simulink model "mu_nonlinear_sim"  (R2026a)
settings: Solver=VariableStepAuto
InitFcn:
  | seaDir=fileparts(get_param(bdroot,'FileName'));if isfile(fullfile(seaDir,'..','collaudo_simulink.m')),addpath(fullfile(seaDir,'..'));else,addpath(fullfile(seaDir,'..','..','File_di_Funzioni_Progetto-Accorpati'));end;collaudo_simulink(bdroot);
undefined symbols (not defined in the file): taubar, xbar
libraries: cstblocks_lti x3
settings Model: Creator=rebec  LastModifiedBy=rebec

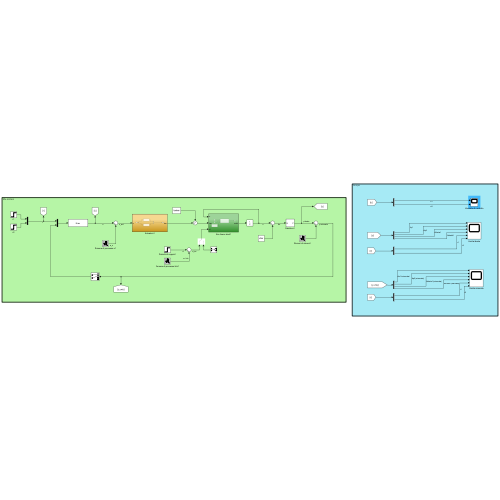
[thumbnail: Simulink's stored preview of the top-level diagram]
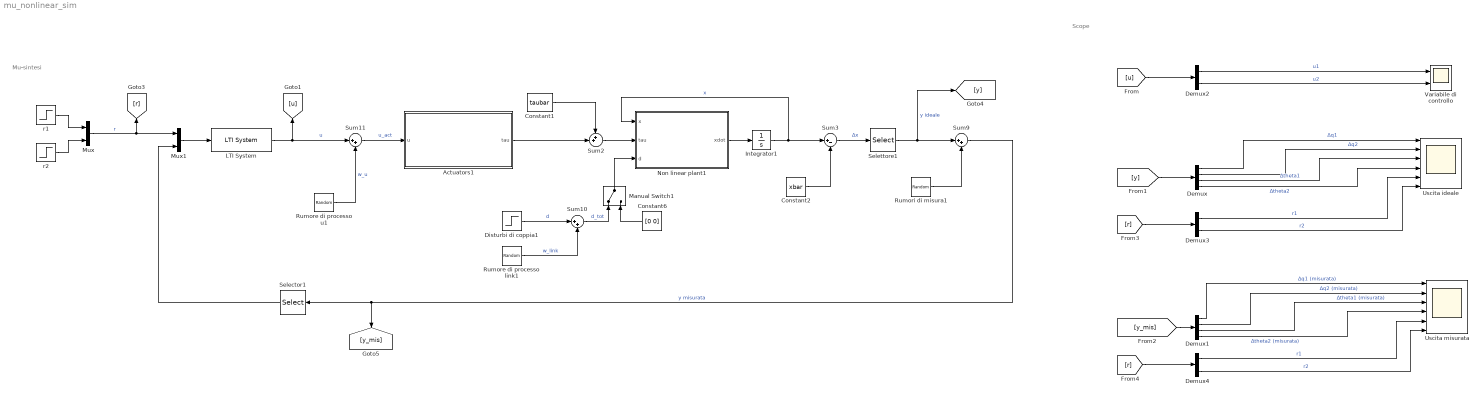
== system mu_nonlinear_sim ==
  note: Scope
  note: Mu-sintesi
  Actuators1 : Subsystem
  Constant1 : Constant  Value=taubar
  Constant2 : Constant  Value=xbar
  Constant6 : Constant  Value=[0 0]
  Demux : Demux
  Demux1 : Demux
  Demux2 : Demux  Outputs=2
  Demux3 : Demux  Outputs=2
  Demux4 : Demux  Outputs=2
  Disturbi di coppia1 : Step  Time=[1 1]  InitialValue=[0 0]  FinalValue=[0.5 0]  SampleTime=0
  Integrator1 : Integrator  InitialCondition=xbar
  LTI System : cstblocks_lti/LTI System  sys=Kmu  IC=[]  PadeOrder=0
      settings: LibrarySourceBlock=cstblocks/LTI System
  Manual Switch1 : ManualSwitch
  Mux : Mux  Inputs=2
  Mux1 : Mux  Inputs=2
  Non linear plant1 : Subsystem
  Rumore di processo link1 : RandomNumber  Mean=[0 0]  Variance=[0.01 0.01]  Seed=20260826  SampleTime=0.002
  Rumore di processo u1 : RandomNumber  Mean=[0 0]  Variance=[0.01 0.01]  Seed=20260826  SampleTime=0.002
  Rumori di misura1 : RandomNumber  Mean=[0 0 0 0]  Variance=[(0.05*pi/180)^2 (0.05*pi/180)^2 (0.05*pi/180)^2 (0.05*pi/180)^2]  Seed=20260826  SampleTime=0.002
  Selector1 : Selector  InputPortWidth=4  IndexOptions=Index vector (dialog)  Indices=[1 2]  OutputSizes=1
  Selettore1 : Selector  InputPortWidth=8  IndexOptions=Index vector (dialog)  Indices=[1 2 5 6]  OutputSizes=1
  Sum10 : Sum  Inputs=|++
  Sum11 : Sum  Inputs=|++
  Sum2 : Sum  Inputs=++|
  Sum3 : Sum  Inputs=|+-
  Sum9 : Sum  Inputs=|++
  Uscita ideale : Scope  NumInputPorts=6
      settings: Title=Uscita ideale (mu NL)  ActiveDisplayYMinimum=-0.088271118920575181  ActiveDisplayYMaximum=0.23303114019935003  YLabel=y (rad)
  Uscita misurata : Scope  NumInputPorts=6
      settings: Title=Uscita misurata (mu NL)  ActiveDisplayYMinimum=-0.11442029066688837  ActiveDisplayYMaximum=0.16914890182413583  YLabel=y (rad)
  Variabile di controllo : Scope  NumInputPorts=2
      settings: Title=Variabili di controllo (mu NL)  ActiveDisplayYMinimum=-14.512240124873713  ActiveDisplayYMaximum=7.6680416810083489  YLabel=u (Nm)  DataLoggingVariableName=ScopeData2
  r1 : Step  FinalValue=5*pi/180  SampleTime=0
  r2 : Step  FinalValue=0  SampleTime=0
  wires:
  Manual Switch1/1 -> Non linear plant1/3(d)
  Selector1/1 -> Mux1/2
  r2/1 -> Mux/2
  Sum9/1 -> [y_mis], Selector1/1  "y misurata"
  r1/1 -> Mux/1
  Integrator1/1 -> Non linear plant1/1(x), Sum3/1  "x"
  Constant2/1 -> Sum3/2
  Sum3/1 -> Selettore1/1  "Δx"
  Sum10/1 -> Manual Switch1/1  "d_tot"
  Constant1/1 -> Sum2/1
  Sum2/1 -> Non linear plant1/2(tau)
  Constant6/1 -> Manual Switch1/2
  Sum11/1 -> Actuators1/1(u)  "u_act"
  Mux/1 -> Mux1/1, [r]  "r"
  Actuators1/1(tau) -> Sum2/2
  Rumore di processo u1/1 -> Sum11/2  "w_u"
  LTI System/1 -> Sum11/1, [u]  "u"
  Selettore1/1 -> Sum9/1, [y]  "y ideale"
  Rumore di processo link1/1 -> Sum10/2  "w_link"
  Disturbi di coppia1/1 -> Sum10/1  "d"
  Mux1/1 -> LTI System/1
  Non linear plant1/1(xdot) -> Integrator1/1
  [y_mis] -> Demux1/1
  Demux4/2 -> Uscita misurata/6  "r2"
  Demux1/4 -> Uscita misurata/4  "Δtheta2 (misurata)"
  [r] -> Demux3/1
  Demux1/2 -> Uscita misurata/2  "Δq2 (misurata)"
  Demux4/1 -> Uscita misurata/5  "r1"
  [r] -> Demux4/1
  Demux/3 -> Uscita ideale/3  "Δtheta1"
  Demux/4 -> Uscita ideale/4  "Δtheta2"
  [y] -> Demux/1
  Demux/1 -> Uscita ideale/1  "Δq1"
  Demux/2 -> Uscita ideale/2  "Δq2"
  Demux2/1 -> Variabile di controllo/1  "u1"
  Demux3/2 -> Uscita ideale/6  "r2"
  Demux1/3 -> Uscita misurata/3  "Δtheta1 (misurata)"
  Demux3/1 -> Uscita ideale/5  "r1"
  Demux2/2 -> Variabile di controllo/2  "u2"
  [u] -> Demux2/1
  Demux1/1 -> Uscita misurata/1  "Δq1 (misurata)"
  Rumori di misura1/1 -> Sum9/2

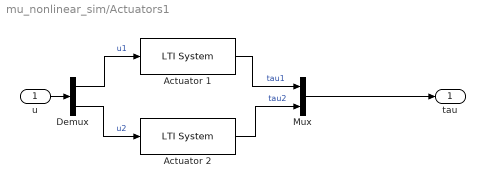
== system mu_nonlinear_sim/Actuators1 ==
  u : Inport
  Actuator 1 : cstblocks_lti/LTI System  sys=Gact  IC=[]  PadeOrder=0
      settings: LibrarySourceBlock=cstblocks/LTI System
  Actuator 2 : cstblocks_lti/LTI System  sys=Gact  IC=[]  PadeOrder=0
      settings: LibrarySourceBlock=cstblocks/LTI System
  Demux : Demux  Outputs=2
  Mux : Mux  Inputs=2
  tau : Outport
  wires:
  Actuator 2/1 -> Mux/2  "tau2"
  Demux/2 -> Actuator 2/1  "u2"
  u/1 -> Demux/1
  Demux/1 -> Actuator 1/1  "u1"
  Mux/1 -> tau/1
  Actuator 1/1 -> Mux/1  "tau1"

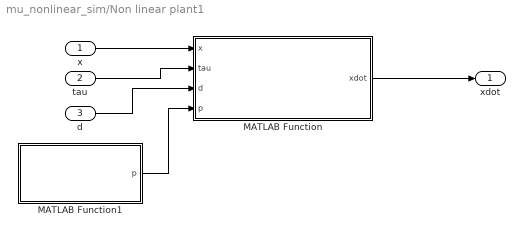
== system mu_nonlinear_sim/Non linear plant1 ==
  x : Inport
  tau : Inport  Port=2
  d : Inport  Port=3
  MATLAB Function : MATLAB Function  TreatAsAtomicUnit=on
  MATLAB Function1 : MATLAB Function  TreatAsAtomicUnit=on
  xdot : Outport
  wires:
  x/1 -> MATLAB Function/1(x)
  tau/1 -> MATLAB Function/2(tau)
  MATLAB Function/1(xdot) -> xdot/1
  MATLAB Function1/1(p) -> MATLAB Function/4(p)
  d/1 -> MATLAB Function/3(d)

== matlab function mu_nonlinear_sim/Non linear plant1/MATLAB Function ==
  data: x input; xdot output; tau input; d input; p input
function xdot = sea_nonlinear_rhs_with_link_disturbance(x, tau, d, p)
%SEA_NONLINEAR_RHS_WITH_LINK_DISTURBANCE SEA dynamics with link torque D.
%   TAU remains the motor-side input; D is an external link-side joint
%   torque entering with positive sign in the link equation.

assert(numel(x) == 8, ...
    'sea_nonlinear_rhs_with_link_disturbance:InvalidState', ...
    'The state must contain exactly eight elements.');
assert(numel(tau) == 2 && numel(d) == 2, ...
    'sea_nonlinear_rhs_with_link_disturbance:InvalidInput', ...
    'Both tau and d must contain exactly two elements.');
x = reshape(x, 8, 1);
tau = reshape(tau, 2, 1);
d = reshape(d, 2, 1);

q = x(1:2);
qdot = x(3:4);
theta = x(5:6);
thetadot = x(7:8);
M = sea_link_inertia(q, p);
C = sea_coriolis(q, qdot, p);
G = sea_gravity(q, p);
tauElastic = sea_elastic_torque(q, theta, p);

qddot = M \ (tauElastic + d - C * qdot - G);
thetaddot = p.Jm \ (tau - p.Bm * thetadot - tauElastic);
xdot = [qdot; qddot; thetadot; thetaddot];
end

== matlab function mu_nonlinear_sim/Non linear plant1/MATLAB Function1 ==
  data: p output Bus: slBus1
function p = sea_params_nominal
%SEA_PARAMS_NOMINAL Nominal mechanical parameters of the 2R SEA robot.
%   P = SEA_PARAMS_NOMINAL returns the values stated by the official
%   assignment. Matrices follow the joint order [joint 1; joint 2].

p.m1 = 1.0;                   % kg
p.m2 = 0.8;                   % kg
p.l1 = 0.4;                   % m
p.l2 = 0.3;                   % m
p.Jm = diag([0.01, 0.01]);    % kg*m^2
p.Bm = diag([0.02, 0.02]);    % N*m*s/rad
p.Ks = diag([50, 40]);        % N*m/rad
p.g = 9.81;                   % m/s^2
end
